simulink model "FMS"  (R2018b)
settings: configuration reference "fms_config" (kept outside this file)
values from neighbouring files (symbols this model uses):
  FMS_EXPORT = Simulink.Parameter(FMS_EXPORT_VALUE)    [fms_model_init.m]
  FMS_PARAM = Simulink.Parameter(FMS_PARAM_VALUE)    [fms_model_init.m]
undefined symbols (not defined in the file or in its folder): actuator_cmd, ax_cmd, ay_cmd, az_cmd, cmd_mask, ControlMode, ctrl_mode, DiscIntNeverNeededParam, ext_state, FMS_Cmd, FMS_CONST, home, mode, p_cmd, phi_cmd, PilotMode, psi_rate_cmd, q_cmd, r_cmd, reset, state, status, theta_cmd, throttle_cmd, timestamp, u_cmd, v_cmd, VehicleState, VehicleStatus, VTOLState, w_cmd, wp_consume, wp_current
libraries: simulink x141, FMT_Model_Lib x120, hdlsllib x13
(part 2 of 12)

== system FMS/FMS Commander/Commander/Arm/FW_Mode/SubMode ==
  In Bus Element{1..5} (5 alike) : Inport  PortName=FMS_In
  Action Port : ActionPort  InitializeStates=reset  ActionType=case
  Bus Selector : BusSelector  OutputSignals=vehicle_state
  Hold : Subsystem
      settings: UndoDeleteFcn=Stateflow.SLINSF.SimulinkMan.restorePreDeleteFcn  PreDeleteFcn=Stateflow.SLINSF.SimulinkMan.removePreDeleteFcn
  Land : Subsystem
      settings: UndoDeleteFcn=Stateflow.SLINSF.SimulinkMan.restorePreDeleteFcn  PreDeleteFcn=Stateflow.SLINSF.SimulinkMan.removePreDeleteFcn
  Merge : Merge  Inputs=5
  Return : Subsystem
      settings: UndoDeleteFcn=Stateflow.SLINSF.SimulinkMan.restorePreDeleteFcn  PreDeleteFcn=Stateflow.SLINSF.SimulinkMan.removePreDeleteFcn
  Switch Case : SwitchCase  CaseConditions={VehicleState.Takeoff, VehicleState.Land, VehicleState.Return,VehicleState.Hold}
  Takeoff : Subsystem
      settings: UndoDeleteFcn=Stateflow.SLINSF.SimulinkMan.restorePreDeleteFcn  PreDeleteFcn=Stateflow.SLINSF.SimulinkMan.removePreDeleteFcn
  Unknown : Subsystem  TreatAsAtomicUnit=on
  FMS_Out : Outport
  wires:
  Merge/1 -> FMS_Out/1
  In Bus Element1/1 -> Land/1(FMS_In)
  Land/1(FMS_Out) -> Merge/2
  Switch Case/2 -> Land/Action
  Switch Case/1 -> Takeoff/Action
  In Bus Element2/1 -> Takeoff/1(FMS_In)
  Takeoff/1(FMS_Out) -> Merge/1
  Switch Case/3 -> Return/Action
  In Bus Element3/1 -> Return/1(FMS_In)
  Return/1(FMS_Out) -> Merge/3
  Hold/1(FMS_Out) -> Merge/4
  In Bus Element4/1 -> Hold/1(FMS_In)
  Switch Case/4 -> Hold/Action
  Switch Case/5 -> Unknown/Action
  Unknown/1(FMS_Out) -> Merge/5
  In Bus Element5/1 -> Bus Selector/1
  Bus Selector/1 -> Switch Case/1  "<vehicle_state>"

== system FMS/FMS Commander/Commander/Arm/FW_Mode/Unknown ==
  Action Port : ActionPort  InitializeStates=reset  ActionType=default
  Bus Assignment : BusAssignment  AssignedSignals=reset,status,state,actuator_cmd
  Constant : Constant  Value=0  OutDataTypeStr=Bus: FMS_Out_Bus
  Constant1 : Constant  Value=VehicleStatus.Disarm
  Constant2 : Constant  OutDataTypeStr=Inherit: Inherit via back propagation
  Constant3 : Constant  Value=[1000;1000;1000;1000]  VectorParams1D=off  OutDataTypeStr=Inherit: Inherit via back propagation
  Constant4 : Constant  Value=zeros(12,1)  OutDataTypeStr=Inherit: Inherit via back propagation
  Constant5 : Constant  Value=VehicleState.Disarm
  Data Type Conversion : DataTypeConversion
  Data Type Conversion1 : DataTypeConversion
  Mux : Mux  Inputs=2
  FMS_Out : Outport
  wires:
  Mux/1 -> Bus Assignment/5
  Constant4/1 -> Mux/2
  Constant3/1 -> Mux/1
  Constant1/1 -> Data Type Conversion/1
  Constant2/1 -> Bus Assignment/2
  Bus Assignment/1 -> FMS_Out/1
  Constant/1 -> Bus Assignment/1
  Constant5/1 -> Data Type Conversion1/1
  Data Type Conversion/1 -> Bus Assignment/3
  Data Type Conversion1/1 -> Bus Assignment/4

== system FMS/FMS Commander/Commander/Arm/MC_Mode/Assist ==
  In Bus Element{1..5} (5 alike) : Inport  PortName=FMS_In
  Action Port : ActionPort  InitializeStates=reset  ActionType=case
  Acro : Subsystem
      settings: UndoDeleteFcn=Stateflow.SLINSF.SimulinkMan.restorePreDeleteFcn  PreDeleteFcn=Stateflow.SLINSF.SimulinkMan.removePreDeleteFcn
  Altitude : Subsystem
      settings: UndoDeleteFcn=Stateflow.SLINSF.SimulinkMan.restorePreDeleteFcn  PreDeleteFcn=Stateflow.SLINSF.SimulinkMan.removePreDeleteFcn
  Bus Selector : BusSelector  OutputSignals=vehicle_state
  Merge : Merge  Inputs=5
  Position : Subsystem
      settings: UndoDeleteFcn=Stateflow.SLINSF.SimulinkMan.restorePreDeleteFcn  PreDeleteFcn=Stateflow.SLINSF.SimulinkMan.removePreDeleteFcn
  Stabilize : Subsystem
      settings: UndoDeleteFcn=Stateflow.SLINSF.SimulinkMan.restorePreDeleteFcn  PreDeleteFcn=Stateflow.SLINSF.SimulinkMan.removePreDeleteFcn
  Switch Case : SwitchCase  CaseConditions={VehicleState.Acro,VehicleState.Stabilize,VehicleState.Altitude,VehicleState.Position}
  Unknown : Subsystem  TreatAsAtomicUnit=on
  FMS_Out : Outport
  wires:
  In Bus Element1/1 -> Position/1(FMS_In)
  Switch Case/4 -> Position/Action
  Switch Case/3 -> Altitude/Action
  In Bus Element2/1 -> Altitude/1(FMS_In)
  Switch Case/2 -> Stabilize/Action
  In Bus Element3/1 -> Stabilize/1(FMS_In)
  In Bus Element4/1 -> Acro/1(FMS_In)
  Switch Case/1 -> Acro/Action
  Acro/1(FMS_Out) -> Merge/1
  Stabilize/1(FMS_Out) -> Merge/2
  Altitude/1(FMS_Out) -> Merge/3
  Position/1(FMS_Out) -> Merge/4
  Merge/1 -> FMS_Out/1
  Unknown/1(FMS_Out) -> Merge/5
  Switch Case/5 -> Unknown/Action
  In Bus Element5/1 -> Bus Selector/1
  Bus Selector/1 -> Switch Case/1  "<vehicle_state>"

== system FMS/FMS Commander/Commander/Arm/MC_Mode/Auto ==
  In Bus Element6 : Inport  PortName=FMS_In
  In Bus Element1 : Inport  PortName=FMS_In
  In Bus Element2 : Inport  PortName=FMS_In
  Action Port : ActionPort  InitializeStates=reset  ActionType=case
  Bus Selector : BusSelector  OutputSignals=vehicle_state
  Merge : Merge  Inputs=3
  Mission : Subsystem
      settings: UndoDeleteFcn=Stateflow.SLINSF.SimulinkMan.restorePreDeleteFcn  PreDeleteFcn=Stateflow.SLINSF.SimulinkMan.removePreDeleteFcn
  Offboard : Subsystem
      settings: UndoDeleteFcn=Stateflow.SLINSF.SimulinkMan.restorePreDeleteFcn  PreDeleteFcn=Stateflow.SLINSF.SimulinkMan.removePreDeleteFcn
  Switch Case : SwitchCase  CaseConditions={VehicleState.Offboard,VehicleState.Mission}
  Unknown : Subsystem  TreatAsAtomicUnit=on
  FMS_Out : Outport
  wires:
  Merge/1 -> FMS_Out/1
  In Bus Element6/1 -> Offboard/1(FMS_In)
  Switch Case/1 -> Offboard/Action
  In Bus Element1/1 -> Mission/1(FMS_In)
  Switch Case/2 -> Mission/Action
  Offboard/1(FMS_Out) -> Merge/1
  Mission/1(FMS_Out) -> Merge/2
  Unknown/1(FMS_Out) -> Merge/3
  Switch Case/3 -> Unknown/Action
  In Bus Element2/1 -> Bus Selector/1
  Bus Selector/1 -> Switch Case/1  "<vehicle_state>"

== system FMS/FMS Commander/Commander/Arm/MC_Mode/Manual ==
  In Bus Element7 : Inport  PortName=FMS_In
  Action Port : ActionPort  InitializeStates=reset  ActionType=case
  Bus Assignment : BusAssignment  AssignedSignals=reset,status,state
  Constant : Constant  Value=0  OutDataTypeStr=Bus: FMS_Out_Bus
  Constant1 : Constant  Value=VehicleStatus.Disarm
  Constant2 : Constant  OutDataTypeStr=Inherit: Inherit via back propagation
  Constant5 : Constant  Value=VehicleState.Manual
  Data Type Conversion : DataTypeConversion
  Data Type Conversion1 : DataTypeConversion
  Terminator : Terminator
  FMS_Out : Outport
  wires:
  Data Type Conversion1/1 -> Bus Assignment/4
  Data Type Conversion/1 -> Bus Assignment/3
  Constant5/1 -> Data Type Conversion1/1
  Constant/1 -> Bus Assignment/1
  Bus Assignment/1 -> FMS_Out/1
  Constant2/1 -> Bus Assignment/2
  Constant1/1 -> Data Type Conversion/1
  In Bus Element7/1 -> Terminator/1

== system FMS/FMS Commander/Commander/Arm/MC_Mode/SubMode ==
  In Bus Element{1..5} (5 alike) : Inport  PortName=FMS_In
  Action Port : ActionPort  InitializeStates=reset  ActionType=case
  Bus Selector : BusSelector  OutputSignals=vehicle_state
  Hold : Subsystem
      settings: UndoDeleteFcn=Stateflow.SLINSF.SimulinkMan.restorePreDeleteFcn  PreDeleteFcn=Stateflow.SLINSF.SimulinkMan.removePreDeleteFcn
  Land : Subsystem
      settings: UndoDeleteFcn=Stateflow.SLINSF.SimulinkMan.restorePreDeleteFcn  PreDeleteFcn=Stateflow.SLINSF.SimulinkMan.removePreDeleteFcn
  Merge : Merge  Inputs=5
  Return : Subsystem
      settings: UndoDeleteFcn=Stateflow.SLINSF.SimulinkMan.restorePreDeleteFcn  PreDeleteFcn=Stateflow.SLINSF.SimulinkMan.removePreDeleteFcn
  Switch Case : SwitchCase  CaseConditions={VehicleState.Takeoff, VehicleState.Land, VehicleState.Return,VehicleState.Hold}
  Takeoff : Subsystem
      settings: UndoDeleteFcn=Stateflow.SLINSF.SimulinkMan.restorePreDeleteFcn  PreDeleteFcn=Stateflow.SLINSF.SimulinkMan.removePreDeleteFcn
  Unknown : Subsystem  TreatAsAtomicUnit=on
  FMS_Out : Outport
  wires:
  Merge/1 -> FMS_Out/1
  In Bus Element1/1 -> Land/1(FMS_In)
  Land/1(FMS_Out) -> Merge/2
  Switch Case/2 -> Land/Action
  Switch Case/1 -> Takeoff/Action
  In Bus Element2/1 -> Takeoff/1(FMS_In)
  Takeoff/1(FMS_Out) -> Merge/1
  Switch Case/3 -> Return/Action
  In Bus Element3/1 -> Return/1(FMS_In)
  Return/1(FMS_Out) -> Merge/3
  Hold/1(FMS_Out) -> Merge/4
  In Bus Element4/1 -> Hold/1(FMS_In)
  Switch Case/4 -> Hold/Action
  Switch Case/5 -> Unknown/Action
  Unknown/1(FMS_Out) -> Merge/5
  In Bus Element5/1 -> Bus Selector/1
  Bus Selector/1 -> Switch Case/1  "<vehicle_state>"

== system FMS/FMS Commander/Commander/Arm/MC_Mode/Unknown ==
  Action Port : ActionPort  InitializeStates=reset  ActionType=default
  Bus Assignment : BusAssignment  AssignedSignals=reset,status,state,actuator_cmd
  Constant : Constant  Value=0  OutDataTypeStr=Bus: FMS_Out_Bus
  Constant1 : Constant  Value=VehicleStatus.Disarm
  Constant2 : Constant  OutDataTypeStr=Inherit: Inherit via back propagation
  Constant3 : Constant  Value=[1000;1000;1000;1000]  VectorParams1D=off  OutDataTypeStr=Inherit: Inherit via back propagation
  Constant4 : Constant  Value=zeros(12,1)  OutDataTypeStr=Inherit: Inherit via back propagation
  Constant5 : Constant  Value=VehicleState.Disarm
  Data Type Conversion : DataTypeConversion
  Data Type Conversion1 : DataTypeConversion
  Mux : Mux  Inputs=2
  FMS_Out : Outport
  wires:
  Mux/1 -> Bus Assignment/5
  Constant4/1 -> Mux/2
  Constant3/1 -> Mux/1
  Constant1/1 -> Data Type Conversion/1
  Constant2/1 -> Bus Assignment/2
  Bus Assignment/1 -> FMS_Out/1
  Constant/1 -> Bus Assignment/1
  Constant5/1 -> Data Type Conversion1/1
  Data Type Conversion/1 -> Bus Assignment/3
  Data Type Conversion1/1 -> Bus Assignment/4

== system FMS/FMS Commander/Commander/Arm/BackwardTrans_Mode/Position Command/Controller ==
  motion_state : Inport
  In Bus Element : Inport  Port=2  PortName=FMS_In
  In Bus Element1 : Inport  Port=2  PortName=FMS_In
  Brake Control : Subsystem  TreatAsAtomicUnit=on
  Hold Control : Subsystem  TreatAsAtomicUnit=on
  Merge : Merge  Inputs=3
  Move Control : Subsystem  TreatAsAtomicUnit=on
  Saturation1 : Saturate  UpperLimit=FMS_PARAM.FW_ACC_Y_LIM  LowerLimit=-FMS_PARAM.FW_ACC_Y_LIM
  Switch Case : SwitchCase  CaseConditions={MotionState.Hold, MotionState.Brake, MotionState.Move}  ShowDefaultCase=off
  ay_cmd_mPs2 : Outport
  wires:
  Move Control/1(ay_cmd_mPs2) -> Merge/3
  Brake Control/1(ay_cmd_mPs2) -> Merge/2
  Hold Control/1(ay_cmd_mPs2) -> Merge/1
  In Bus Element/1 -> Hold Control/1(FMS_In)
  Switch Case/3 -> Move Control/Action
  Switch Case/2 -> Brake Control/Action
  Switch Case/1 -> Hold Control/Action
  motion_state/1 -> Switch Case/1
  Saturation1/1 -> ay_cmd_mPs2/1
  Merge/1 -> Saturation1/1
  In Bus Element1/1 -> Move Control/1(FMS_In)

== system FMS/FMS Commander/Commander/Arm/BackwardTrans_Mode/Position Command/Detect Movement ==
  FMS_In : Inport
  Abs : Abs
  Abs1 : Abs
  Abs2 : Abs
  Bus Selector1 : BusSelector  OutputSignals=Pilot_Cmd.stick_roll,Pilot_Cmd.stick_yaw
  Bus Selector2 : BusSelector  OutputSignals=INS_Out.psi,INS_Out.vn,INS_Out.ve,INS_Out.vd
  Compare To Constant : simulink/Logic and Bit Operations/Compare To Constant  relop=>  const=FMS_PARAM.ROLL_DZ  OutDataTypeStr=boolean
  Compare To Constant1 : simulink/Logic and Bit Operations/Compare To Constant  relop=>  const=FMS_PARAM.YAW_DZ  OutDataTypeStr=boolean
  Logical Operator : Logic  Operator=OR  AllPortsSameDT=off  OutDataTypeStr=boolean
  Motion State : Stateflow chart  TreatAsAtomicUnit=on
  Multiply : Product  Multiplication=Matrix(*)
  Mux : Mux  Inputs=3
  Psi To DCM : FMT_Model_Lib/Transformation/Psi To DCM
      settings: SourceProductName=FMT Toolbox
  Selector : Selector  InputPortWidth=3  IndexOptions=Index vector (dialog)  Indices=1  OutputSizes=1
  motion_state : Outport
  wires:
  FMS_In/1 -> Bus Selector2/1, Bus Selector1/1
  Abs1/1 -> Compare To Constant/1
  Motion State/1(state) -> motion_state/1
  Abs/1 -> Motion State/2(speed)
  Bus Selector1/1 -> Abs1/1  "<stick_roll>"
  Bus Selector2/1 -> Psi To DCM/1  "<psi>"
  Bus Selector2/2 -> Mux/1  "<vn>"
  Bus Selector2/3 -> Mux/2  "<ve>"
  Bus Selector2/4 -> Mux/3  "<vd>"
  Psi To DCM/1 -> Multiply/1
  Multiply/1 -> Selector/1
  Selector/1 -> Abs/1
  Mux/1 -> Multiply/2
  Bus Selector1/2 -> Abs2/1  "<stick_yaw>"
  Abs2/1 -> Compare To Constant1/1
  Compare To Constant/1 -> Logical Operator/1
  Compare To Constant1/1 -> Logical Operator/2
  Logical Operator/1 -> Motion State/1(motion_req)

== system FMS/FMS Commander/Commander/Arm/BackwardTrans_Mode/mapping/DeadZone ==
  u : Inport
  Dead Zone : DeadZone  LowerValue=-th  UpperValue=th  SaturateOnIntegerOverflow=on
  Gain : Gain  Gain=1/(1-th)
  y : Outport
  wires:
  Gain/1 -> y/1
  Dead Zone/1 -> Gain/1
  u/1 -> Dead Zone/1

== system FMS/FMS Commander/Commander/Arm/BackwardTrans_Mode/mapping/DeadZone1 ==
  u : Inport
  Dead Zone : DeadZone  LowerValue=-th  UpperValue=th  SaturateOnIntegerOverflow=on
  Gain : Gain  Gain=1/(1-th)
  y : Outport
  wires:
  u/1 -> Dead Zone/1
  Dead Zone/1 -> Gain/1
  Gain/1 -> y/1

== system FMS/FMS Commander/Commander/Arm/BackwardTrans_Mode/mapping/DeadZone2 ==
  u : Inport
  Dead Zone : DeadZone  LowerValue=-th  UpperValue=th  SaturateOnIntegerOverflow=on
  Gain : Gain  Gain=1/(1-th)
  y : Outport
  wires:
  Gain/1 -> y/1
  Dead Zone/1 -> Gain/1
  u/1 -> Dead Zone/1

== system FMS/FMS Commander/Commander/Arm/BackwardTrans_Mode/mapping/TD ==
  v : Inport
  Integrator : DiscreteIntegrator  SampleTime=-1  ICPrevOutput=DiscIntNeverNeededParam  ICPrevScaledInput=DiscIntNeverNeededParam
  Integrator1 : DiscreteIntegrator  SampleTime=-1  ICPrevOutput=DiscIntNeverNeededParam  ICPrevScaledInput=DiscIntNeverNeededParam
  Signal Copy : SignalConversion  OverrideOpt=off
  Subtract : Sum  Inputs=+-
  "fhan " : Subsystem  mask{r0=4*9.806, h0=0.1}
      mask DialogControl ParameterGroupVar Prompt: fhan(v1,v2,r0,h0)
  v1 : Outport
  wires:
  "fhan "/1(fhan) -> Integrator/1
  Subtract/1 -> "fhan "/1(v1)
  Integrator/1 -> Integrator1/1, "fhan "/2(v2)  "v2"
  v/1 -> Subtract/2
  Integrator1/1 -> Subtract/1, Signal Copy/1
  Signal Copy/1 -> v1/1

== system FMS/FMS Commander/Commander/Arm/BackwardTrans_Mode/mapping/TD1 ==
  v : Inport
  Integrator : DiscreteIntegrator  SampleTime=-1  ICPrevOutput=DiscIntNeverNeededParam  ICPrevScaledInput=DiscIntNeverNeededParam
  Integrator1 : DiscreteIntegrator  SampleTime=-1  ICPrevOutput=DiscIntNeverNeededParam  ICPrevScaledInput=DiscIntNeverNeededParam
  Signal Copy : SignalConversion  OverrideOpt=off
  Subtract : Sum  Inputs=+-
  "fhan " : Subsystem  mask{r0=5*pi, h0=0.02}
      mask DialogControl ParameterGroupVar Prompt: fhan(v1,v2,r0,h0)
  v1 : Outport
  wires:
  "fhan "/1(fhan) -> Integrator/1
  Subtract/1 -> "fhan "/1(v1)
  Integrator/1 -> Integrator1/1, "fhan "/2(v2)  "v2"
  v/1 -> Subtract/2
  Integrator1/1 -> Subtract/1, Signal Copy/1
  Signal Copy/1 -> v1/1

== system FMS/FMS Commander/Commander/Arm/BackwardTrans_Mode/mapping/TD2 ==
  v : Inport
  Integrator : DiscreteIntegrator  SampleTime=-1  ICPrevOutput=DiscIntNeverNeededParam  ICPrevScaledInput=DiscIntNeverNeededParam
  Integrator1 : DiscreteIntegrator  SampleTime=-1  ICPrevOutput=DiscIntNeverNeededParam  ICPrevScaledInput=DiscIntNeverNeededParam
  Signal Copy : SignalConversion  OverrideOpt=off
  Subtract : Sum  Inputs=+-
  "fhan " : Subsystem  mask{r0=4*9.806, h0=0.1}
      mask DialogControl ParameterGroupVar Prompt: fhan(v1,v2,r0,h0)
  v1 : Outport
  wires:
  Signal Copy/1 -> v1/1
  Integrator1/1 -> Signal Copy/1, Subtract/1
  v/1 -> Subtract/2
  Integrator/1 -> "fhan "/2(v2), Integrator1/1  "v2"
  Subtract/1 -> "fhan "/1(v1)
  "fhan "/1(fhan) -> Integrator/1

== system FMS/FMS Commander/Commander/Arm/FW_Mode/Assist/Altitude ==
  In Bus Element1 : Inport  PortName=FMS_In
  Action Port : ActionPort  InitializeStates=reset  ActionType=case
      settings: CopyFcn=Stateflow.SLINSF.SimulinkMan.removeBlockPreDeleteFcn
  Altitude Command : Subsystem
  Attitude Command : Subsystem
  Bus Assignment : BusAssignment  AssignedSignals=status,state,ctrl_mode,phi_cmd,psi_rate_cmd,u_cmd,w_cmd
  Constant : Constant  Value=0  OutDataTypeStr=Bus: FMS_Out_Bus
  Constant1 : Constant  Value=VehicleState.Altitude
  Constant2 : Constant  Value=ControlMode.ALTCTL
  Constant5 : Constant  Value=VehicleStatus.Arm
  Data Type Conversion1 : DataTypeConversion
  Data Type Conversion2 : DataTypeConversion
  Data Type Conversion3 : DataTypeConversion
  Heading Command : Subsystem
  Speed Command : Subsystem
  FMS_Out : Outport
  wires:
  Constant5/1 -> Data Type Conversion1/1
  Constant/1 -> Bus Assignment/1
  Altitude Command/1(w_cmd_mPs) -> Bus Assignment/8
  Attitude Command/1(phi_cmd_radPs) -> Bus Assignment/5
  Bus Assignment/1 -> FMS_Out/1
  Data Type Conversion1/1 -> Bus Assignment/2
  Constant1/1 -> Data Type Conversion2/1
  Data Type Conversion2/1 -> Bus Assignment/3
  Data Type Conversion3/1 -> Bus Assignment/4
  Constant2/1 -> Data Type Conversion3/1
  In Bus Element1/1 -> Heading Command/1(FMS_In), Attitude Command/1(FMS_In), Speed Command/1(FMS_In), Altitude Command/1(FMS_In)
  Speed Command/1(u_cmd_mPs) -> Bus Assignment/7
  Heading Command/1(psi_rate_cmd_radPs) -> Bus Assignment/6

== system FMS/FMS Commander/Commander/Arm/FW_Mode/Assist/Position ==
  FMS_In : Inport
  Action Port : ActionPort  InitializeStates=reset  ActionType=case
      settings: CopyFcn=Stateflow.SLINSF.SimulinkMan.removeBlockPreDeleteFcn
  Altitude Command : Subsystem
  Bus Assignment : BusAssignment  AssignedSignals=status,state,ctrl_mode,psi_rate_cmd,u_cmd,ay_cmd,w_cmd
  Constant : Constant  Value=0  OutDataTypeStr=Bus: FMS_Out_Bus
  Constant1 : Constant  Value=VehicleState.Position
  Constant2 : Constant  Value=ControlMode.POSCTL
  Constant5 : Constant  Value=VehicleStatus.Arm
  Data Type Conversion : DataTypeConversion
  Data Type Conversion1 : DataTypeConversion
  Data Type Conversion2 : DataTypeConversion
  Heading Command : Subsystem
  Position Command : Subsystem
  Speed Command : Subsystem
  FMS_Out : Outport
  wires:
  Bus Assignment/1 -> FMS_Out/1
  Altitude Command/1(w_cmd_mPs) -> Bus Assignment/8
  Constant/1 -> Bus Assignment/1
  Constant5/1 -> Data Type Conversion/1
  Position Command/1(ay_cmd_mPs2) -> Bus Assignment/7
  Data Type Conversion/1 -> Bus Assignment/2
  Constant1/1 -> Data Type Conversion1/1
  Data Type Conversion1/1 -> Bus Assignment/3
  Constant2/1 -> Data Type Conversion2/1
  Data Type Conversion2/1 -> Bus Assignment/4
  FMS_In/1 -> Altitude Command/1(FMS_In), Position Command/1(FMS_In), Heading Command/1(FMS_In), Speed Command/1(FMS_In)
  Speed Command/1(u_cmd_mPs) -> Bus Assignment/6
  Heading Command/1(psi_rate_cmd_radPs) -> Bus Assignment/5

== system FMS/FMS Commander/Commander/Arm/FW_Mode/Assist/Stabilize ==
  FMS_In : Inport
  Action Port : ActionPort  InitializeStates=reset  ActionType=case
      settings: CopyFcn=Stateflow.SLINSF.SimulinkMan.removeBlockPreDeleteFcn
  Attitude Command : Subsystem
  Bus Assignment : BusAssignment  AssignedSignals=status,state,ctrl_mode,phi_cmd,theta_cmd,psi_rate_cmd,throttle_cmd
  Constant : Constant  Value=0  OutDataTypeStr=Bus: FMS_Out_Bus
  Constant1 : Constant  Value=VehicleState.Stabilize
  Constant2 : Constant  Value=ControlMode.Stabilize
  Constant5 : Constant  Value=VehicleStatus.Arm
  Data Type Conversion : DataTypeConversion
  Data Type Conversion1 : DataTypeConversion
  Data Type Conversion2 : DataTypeConversion
  Heading Command : Subsystem
  Throttle Command : Subsystem
  FMS_Out : Outport
  wires:
  Constant5/1 -> Data Type Conversion/1
  Constant/1 -> Bus Assignment/1
  Attitude Command/1(phi_cmd_radPs) -> Bus Assignment/5
  Throttle Command/1(throttle_cmd) -> Bus Assignment/8
  Attitude Command/2(theta_cmd_radPs) -> Bus Assignment/6
  FMS_In/1 -> Heading Command/1(FMS_In), Throttle Command/1(FMS_In), Attitude Command/1(FMS_In)
  Bus Assignment/1 -> FMS_Out/1
  Data Type Conversion/1 -> Bus Assignment/2
  Constant1/1 -> Data Type Conversion1/1
  Data Type Conversion1/1 -> Bus Assignment/3
  Constant2/1 -> Data Type Conversion2/1
  Data Type Conversion2/1 -> Bus Assignment/4
  Heading Command/1(psi_rate_cmd_radPs) -> Bus Assignment/7

== system FMS/FMS Commander/Commander/Arm/FW_Mode/Assist/Unknown ==
  Action Port : ActionPort  InitializeStates=reset  ActionType=default
  Bus Assignment : BusAssignment  AssignedSignals=reset,status,state,actuator_cmd
  Constant : Constant  Value=0  OutDataTypeStr=Bus: FMS_Out_Bus
  Constant1 : Constant  Value=VehicleStatus.Disarm
  Constant2 : Constant  OutDataTypeStr=Inherit: Inherit via back propagation
  Constant3 : Constant  Value=[1000;1000;1000;1000]  VectorParams1D=off  OutDataTypeStr=Inherit: Inherit via back propagation
  Constant4 : Constant  Value=zeros(12,1)  OutDataTypeStr=Inherit: Inherit via back propagation
  Constant5 : Constant  Value=VehicleState.Disarm
  Data Type Conversion : DataTypeConversion
  Data Type Conversion1 : DataTypeConversion
  Mux : Mux  Inputs=2
  FMS_Out : Outport
  wires:
  Mux/1 -> Bus Assignment/5
  Constant4/1 -> Mux/2
  Constant3/1 -> Mux/1
  Constant1/1 -> Data Type Conversion/1
  Constant2/1 -> Bus Assignment/2
  Bus Assignment/1 -> FMS_Out/1
  Constant/1 -> Bus Assignment/1
  Constant5/1 -> Data Type Conversion1/1
  Data Type Conversion/1 -> Bus Assignment/3
  Data Type Conversion1/1 -> Bus Assignment/4

== system FMS/FMS Commander/Commander/Arm/FW_Mode/Auto/Mission ==
  FMS_In : Inport
  Action Port : ActionPort  InitializeStates=reset  ActionType=case
      settings: CopyFcn=Stateflow.SLINSF.SimulinkMan.removeBlockPreDeleteFcn
  Bus Selector : BusSelector  OutputSignals=wp_index
  Detect Change : simulink/Logic and Bit Operations/Detect Change  vinit=0  OutDataTypeStr=boolean
  Mission_SubSystem : Subsystem  TreatAsAtomicUnit=on
  FMS_Out : Outport
  wires:
  Mission_SubSystem/1(FMS_Out) -> FMS_Out/1
  FMS_In/1 -> Bus Selector/1, Mission_SubSystem/1(FMS_In)
  Bus Selector/1 -> Detect Change/1  "<wp_index>"
  Detect Change/1 -> Mission_SubSystem/Reset

== system FMS/FMS Commander/Commander/Arm/FW_Mode/Auto/Offboard ==
  FMS_In : Inport
  Action Port : ActionPort  InitializeStates=reset  ActionType=case
      settings: CopyFcn=Stateflow.SLINSF.SimulinkMan.removeBlockPreDeleteFcn
  Bus Assignment : BusAssignment  AssignedSignals=status,state
  Constant : Constant  Value=0  OutDataTypeStr=Bus: FMS_Out_Bus
  Constant1 : Constant  Value=VehicleStatus.Disarm
  Constant2 : Constant  Value=VehicleState.Offboard
  Data Type Conversion : DataTypeConversion
  Data Type Conversion1 : DataTypeConversion
  Terminator : Terminator
  FMS_Out : Outport
  wires:
  Bus Assignment/1 -> FMS_Out/1
  Constant/1 -> Bus Assignment/1
  FMS_In/1 -> Terminator/1
  Constant1/1 -> Data Type Conversion/1
  Data Type Conversion/1 -> Bus Assignment/2
  Constant2/1 -> Data Type Conversion1/1
  Data Type Conversion1/1 -> Bus Assignment/3

== system FMS/FMS Commander/Commander/Arm/FW_Mode/Auto/Unknown ==
  Action Port : ActionPort  InitializeStates=reset  ActionType=default
  Bus Assignment : BusAssignment  AssignedSignals=reset,status,state,actuator_cmd
  Constant : Constant  Value=0  OutDataTypeStr=Bus: FMS_Out_Bus
  Constant1 : Constant  Value=VehicleStatus.Disarm
  Constant2 : Constant  OutDataTypeStr=Inherit: Inherit via back propagation
  Constant3 : Constant  Value=[1000;1000;1000;1000]  VectorParams1D=off  OutDataTypeStr=Inherit: Inherit via back propagation
  Constant4 : Constant  Value=zeros(12,1)  OutDataTypeStr=Inherit: Inherit via back propagation
  Constant5 : Constant  Value=VehicleState.Disarm
  Data Type Conversion : DataTypeConversion
  Data Type Conversion1 : DataTypeConversion
  Mux : Mux  Inputs=2
  FMS_Out : Outport
  wires:
  Mux/1 -> Bus Assignment/5
  Constant4/1 -> Mux/2
  Constant3/1 -> Mux/1
  Constant1/1 -> Data Type Conversion/1
  Constant2/1 -> Bus Assignment/2
  Bus Assignment/1 -> FMS_Out/1
  Constant/1 -> Bus Assignment/1
  Constant5/1 -> Data Type Conversion1/1
  Data Type Conversion/1 -> Bus Assignment/3
  Data Type Conversion1/1 -> Bus Assignment/4

== system FMS/FMS Commander/Commander/Arm/FW_Mode/Manual/DeadZone ==
  u : Inport
  Dead Zone : DeadZone  LowerValue=-th  UpperValue=th  SaturateOnIntegerOverflow=on
  Gain : Gain  Gain=1/(1-th)
  y : Outport
  wires:
  Gain/1 -> y/1
  Dead Zone/1 -> Gain/1
  u/1 -> Dead Zone/1

== system FMS/FMS Commander/Commander/Arm/FW_Mode/Manual/DeadZone1 ==
  u : Inport
  Dead Zone : DeadZone  LowerValue=-th  UpperValue=th  SaturateOnIntegerOverflow=on
  Gain : Gain  Gain=1/(1-th)
  y : Outport
  wires:
  u/1 -> Dead Zone/1
  Dead Zone/1 -> Gain/1
  Gain/1 -> y/1

== system FMS/FMS Commander/Commander/Arm/FW_Mode/Manual/DeadZone2 ==
  u : Inport
  Dead Zone : DeadZone  LowerValue=-th  UpperValue=th  SaturateOnIntegerOverflow=on
  Gain : Gain  Gain=1/(1-th)
  y : Outport
  wires:
  Gain/1 -> y/1
  Dead Zone/1 -> Gain/1
  u/1 -> Dead Zone/1

== system FMS/FMS Commander/Commander/Arm/FW_Mode/Manual/DeadZone3 ==
  u : Inport
  Dead Zone : DeadZone  LowerValue=-th  UpperValue=th  SaturateOnIntegerOverflow=on
  Gain : Gain  Gain=1/(1-th)
  y : Outport
  wires:
  u/1 -> Dead Zone/1
  Dead Zone/1 -> Gain/1
  Gain/1 -> y/1

== system FMS/FMS Commander/Commander/Arm/FW_Mode/SubMode/Hold ==
  FMS_In : Inport
  Action Port : ActionPort  InitializeStates=reset  ActionType=case
      settings: CopyFcn=Stateflow.SLINSF.SimulinkMan.removeBlockPreDeleteFcn
  Altitude_Hold : Subsystem
  Bus Assignment : BusAssignment  AssignedSignals=status,state,ctrl_mode,u_cmd,ay_cmd,w_cmd
  Constant : Constant  Value=0  OutDataTypeStr=Bus: FMS_Out_Bus
  Constant1 : Constant  Value=VehicleState.Hold
  Constant2 : Constant  Value=ControlMode.POSCTL
  Constant3 : Constant  Value=15  OutDataTypeStr=single
  Constant5 : Constant  Value=VehicleStatus.Arm
  Data Type Conversion : DataTypeConversion
  Data Type Conversion1 : DataTypeConversion
  Data Type Conversion2 : DataTypeConversion
  Loiter_Control : Subsystem
  FMS_Out : Outport
  wires:
  Bus Assignment/1 -> FMS_Out/1
  Altitude_Hold/1(w_cmd_mPs) -> Bus Assignment/7
  Constant/1 -> Bus Assignment/1
  Constant5/1 -> Data Type Conversion/1
  Data Type Conversion/1 -> Bus Assignment/2
  Constant1/1 -> Data Type Conversion1/1
  Data Type Conversion1/1 -> Bus Assignment/3
  Constant2/1 -> Data Type Conversion2/1
  Data Type Conversion2/1 -> Bus Assignment/4
  FMS_In/1 -> Altitude_Hold/1(FMS_In), Loiter_Control/1(FMS_In)
  Loiter_Control/1(ay_cmd_mPs2) -> Bus Assignment/6
  Constant3/1 -> Bus Assignment/5

== system FMS/FMS Commander/Commander/Arm/FW_Mode/SubMode/Land ==
  FMS_In : Inport
  Action Port : ActionPort  InitializeStates=reset  ActionType=case
      settings: CopyFcn=Stateflow.SLINSF.SimulinkMan.removeBlockPreDeleteFcn
  Bus Assignment1 : BusAssignment  AssignedSignals=status,state,ctrl_mode,psi_rate_cmd,u_cmd,v_cmd,w_cmd
  Constant : Constant  Value=0  OutDataTypeStr=Inherit: Inherit via back propagation
  Constant1 : Constant  Value=0  OutDataTypeStr=Bus: FMS_Out_Bus
  Constant2 : Constant  Value=ControlMode.POSCTL
  Constant3 : Constant  Value=VehicleState.Land
  Constant4 : Constant  Value=0.5  OutDataTypeStr=Inherit: Inherit via back propagation
  Constant5 : Constant  Value=0  OutDataTypeStr=Inherit: Inherit via back propagation
  Constant6 : Constant  Value=VehicleStatus.Arm
  Constant7 : Constant  Value=0  OutDataTypeStr=Inherit: Inherit via back propagation
  Data Type Conversion : DataTypeConversion
  Data Type Conversion1 : DataTypeConversion
  Data Type Conversion2 : DataTypeConversion
  Terminator : Terminator
  FMS_Out : Outport
  wires:
  Bus Assignment1/1 -> FMS_Out/1
  Constant1/1 -> Bus Assignment1/1
  FMS_In/1 -> Terminator/1
  Constant4/1 -> Bus Assignment1/8
  Constant/1 -> Bus Assignment1/5
  Constant2/1 -> Data Type Conversion2/1
  Constant6/1 -> Data Type Conversion/1
  Data Type Conversion/1 -> Bus Assignment1/2
  Constant3/1 -> Data Type Conversion1/1
  Data Type Conversion1/1 -> Bus Assignment1/3
  Data Type Conversion2/1 -> Bus Assignment1/4
  Constant5/1 -> Bus Assignment1/6
  Constant7/1 -> Bus Assignment1/7

== system FMS/FMS Commander/Commander/Arm/FW_Mode/SubMode/Return ==
  FMS_In : Inport
  Action Port : ActionPort  InitializeStates=reset  ActionType=case
      settings: CopyFcn=Stateflow.SLINSF.SimulinkMan.removeBlockPreDeleteFcn
  Altitude Control : Subsystem
  Bus Assignment1 : BusAssignment  AssignedSignals=status,state,ctrl_mode,u_cmd,ay_cmd,w_cmd
  Constant1 : Constant  Value=VehicleState.Return
  Constant2 : Constant  Value=0  OutDataTypeStr=Bus: FMS_Out_Bus
  Constant3 : Constant  Value=ControlMode.POSCTL
  Constant4 : Constant  Value=FMS_PARAM.FW_CRUISE_SPEED
  Constant6 : Constant  Value=VehicleStatus.Arm
  Data Type Conversion : DataTypeConversion
  Data Type Conversion1 : DataTypeConversion
  Data Type Conversion2 : DataTypeConversion
  Position Command : Subsystem
  FMS_Out : Outport
  wires:
  Constant3/1 -> Data Type Conversion2/1
  Constant2/1 -> Bus Assignment1/1
  Bus Assignment1/1 -> FMS_Out/1
  Data Type Conversion/1 -> Bus Assignment1/2
  Constant6/1 -> Data Type Conversion/1
  Data Type Conversion1/1 -> Bus Assignment1/3
  Data Type Conversion2/1 -> Bus Assignment1/4
  Constant1/1 -> Data Type Conversion1/1
  FMS_In/1 -> Altitude Control/1(FMS_In), Position Command/1(FMS_In)
  Position Command/1(ay_cmd_mPs2) -> Bus Assignment1/6
  Constant4/1 -> Bus Assignment1/5
  Altitude Control/1(w_cmd_mPs) -> Bus Assignment1/7

== system FMS/FMS Commander/Commander/Arm/FW_Mode/SubMode/Takeoff ==
  FMS_In : Inport
  Action Port : ActionPort  InitializeStates=reset  ActionType=case
      settings: CopyFcn=Stateflow.SLINSF.SimulinkMan.removeBlockPreDeleteFcn
  Altitude Control : Subsystem
  Bus Assignment : BusAssignment  AssignedSignals=status,state,ctrl_mode,u_cmd,ay_cmd,w_cmd
  Constant : Constant  Value=0  OutDataTypeStr=Bus: FMS_Out_Bus
  Constant1 : Constant  Value=VehicleStatus.Arm
  Constant2 : Constant  Value=VehicleState.Takeoff
  Constant3 : Constant  Value=ControlMode.POSCTL
  Constant4 : Constant  Value=FMS_PARAM.FW_CRUISE_SPEED
  Data Type Conversion : DataTypeConversion
  Data Type Conversion1 : DataTypeConversion
  Data Type Conversion2 : DataTypeConversion
  Position Command : Subsystem
  FMS_Out : Outport
  wires:
  Data Type Conversion1/1 -> Bus Assignment/3
  Bus Assignment/1 -> FMS_Out/1
  Constant1/1 -> Data Type Conversion/1
  Constant/1 -> Bus Assignment/1
  Data Type Conversion2/1 -> Bus Assignment/4
  FMS_In/1 -> Altitude Control/1(FMS_In), Position Command/1(FMS_In)
  Data Type Conversion/1 -> Bus Assignment/2
  Constant3/1 -> Data Type Conversion2/1
  Position Command/1(ay_cmd_mPs2) -> Bus Assignment/6
  Constant2/1 -> Data Type Conversion1/1
  Altitude Control/1(w_cmd_mPs) -> Bus Assignment/7
  Constant4/1 -> Bus Assignment/5

== system FMS/FMS Commander/Commander/Arm/FW_Mode/SubMode/Unknown ==
  Action Port : ActionPort  InitializeStates=reset  ActionType=default
  Bus Assignment : BusAssignment  AssignedSignals=reset,status,state,actuator_cmd
  Constant : Constant  Value=0  OutDataTypeStr=Bus: FMS_Out_Bus
  Constant1 : Constant  Value=VehicleStatus.Disarm
  Constant2 : Constant  OutDataTypeStr=Inherit: Inherit via back propagation
  Constant3 : Constant  Value=[1000;1000;1000;1000]  VectorParams1D=off  OutDataTypeStr=Inherit: Inherit via back propagation
  Constant4 : Constant  Value=zeros(12,1)  OutDataTypeStr=Inherit: Inherit via back propagation
  Constant5 : Constant  Value=VehicleState.Disarm
  Data Type Conversion : DataTypeConversion
  Data Type Conversion1 : DataTypeConversion
  Mux : Mux  Inputs=2
  FMS_Out : Outport
  wires:
  Mux/1 -> Bus Assignment/5
  Constant4/1 -> Mux/2
  Constant3/1 -> Mux/1
  Constant1/1 -> Data Type Conversion/1
  Constant2/1 -> Bus Assignment/2
  Bus Assignment/1 -> FMS_Out/1
  Constant/1 -> Bus Assignment/1
  Constant5/1 -> Data Type Conversion1/1
  Data Type Conversion/1 -> Bus Assignment/3
  Data Type Conversion1/1 -> Bus Assignment/4

== system FMS/FMS Commander/Commander/Arm/MC_Mode/Assist/Acro ==
  FMS_In : Inport
  Action Port : ActionPort  InitializeStates=reset  ActionType=case
      settings: CopyFcn=Stateflow.SLINSF.SimulinkMan.removeBlockPreDeleteFcn
  Angular Rate Command : Subsystem
  Bus Assignment : BusAssignment  AssignedSignals=status,state,ctrl_mode,p_cmd,q_cmd,r_cmd,throttle_cmd
  Constant : Constant  Value=0  OutDataTypeStr=Bus: FMS_Out_Bus
  Constant1 : Constant  Value=VehicleState.Acro
  Constant2 : Constant  Value=ControlMode.Acro
  Constant5 : Constant  Value=VehicleStatus.Arm
  Data Type Conversion : DataTypeConversion
  Data Type Conversion1 : DataTypeConversion
  Data Type Conversion2 : DataTypeConversion
  Throttle Command : Subsystem
  FMS_Out : Outport
  wires:
  Data Type Conversion2/1 -> Bus Assignment/4
  Constant2/1 -> Data Type Conversion2/1
  Data Type Conversion1/1 -> Bus Assignment/3
  Constant1/1 -> Data Type Conversion1/1
  Data Type Conversion/1 -> Bus Assignment/2
  Bus Assignment/1 -> FMS_Out/1
  Throttle Command/1(throttle_cmd) -> Bus Assignment/8
  Constant/1 -> Bus Assignment/1
  Constant5/1 -> Data Type Conversion/1
  Angular Rate Command/1(p_cmd_radPs) -> Bus Assignment/5
  Angular Rate Command/2(q_cmd_radPs) -> Bus Assignment/6
  Angular Rate Command/3(r_cmd_radPs) -> Bus Assignment/7
  FMS_In/1 -> Throttle Command/1(FMS_In), Angular Rate Command/1(FMS_In)

== system FMS/FMS Commander/Commander/Arm/MC_Mode/Assist/Altitude ==
  In Bus Element1 : Inport  PortName=FMS_In
  Action Port : ActionPort  InitializeStates=reset  ActionType=case
      settings: CopyFcn=Stateflow.SLINSF.SimulinkMan.removeBlockPreDeleteFcn
  Altitude Command : Subsystem
  Attitude Command : Subsystem
  Bus Assignment : BusAssignment  AssignedSignals=status,state,ctrl_mode,phi_cmd,theta_cmd,psi_rate_cmd,w_cmd
  Constant : Constant  Value=0  OutDataTypeStr=Bus: FMS_Out_Bus
  Constant1 : Constant  Value=VehicleState.Altitude
  Constant2 : Constant  Value=ControlMode.ALTCTL
  Constant5 : Constant  Value=VehicleStatus.Arm
  Data Type Conversion1 : DataTypeConversion
  Data Type Conversion2 : DataTypeConversion
  Data Type Conversion3 : DataTypeConversion
  Heading Command : Subsystem
  FMS_Out : Outport
  wires:
  Constant5/1 -> Data Type Conversion1/1
  Constant/1 -> Bus Assignment/1
  Heading Command/1(psi_rate_cmd_radPs) -> Bus Assignment/7
  Altitude Command/1(w_cmd_mPs) -> Bus Assignment/8
  Attitude Command/1(phi_cmd_radPs) -> Bus Assignment/5
  Attitude Command/2(theta_cmd_radPs) -> Bus Assignment/6
  Bus Assignment/1 -> FMS_Out/1
  Data Type Conversion1/1 -> Bus Assignment/2
  Constant1/1 -> Data Type Conversion2/1
  Data Type Conversion2/1 -> Bus Assignment/3
  Data Type Conversion3/1 -> Bus Assignment/4
  Constant2/1 -> Data Type Conversion3/1
  In Bus Element1/1 -> Heading Command/1(FMS_In), Altitude Command/1(FMS_In), Attitude Command/1(FMS_In)

== system FMS/FMS Commander/Commander/Arm/MC_Mode/Assist/Position ==
  FMS_In : Inport
  Action Port : ActionPort  InitializeStates=reset  ActionType=case
      settings: CopyFcn=Stateflow.SLINSF.SimulinkMan.removeBlockPreDeleteFcn
  Altitude Command : Subsystem
  Bus Assignment : BusAssignment  AssignedSignals=status,state,ctrl_mode,psi_rate_cmd,u_cmd,v_cmd,w_cmd
  Constant : Constant  Value=0  OutDataTypeStr=Bus: FMS_Out_Bus
  Constant1 : Constant  Value=VehicleState.Position
  Constant2 : Constant  Value=ControlMode.POSCTL
  Constant5 : Constant  Value=VehicleStatus.Arm
  Data Type Conversion : DataTypeConversion
  Data Type Conversion1 : DataTypeConversion
  Data Type Conversion2 : DataTypeConversion
  Heading Command : Subsystem
  Position Command : Subsystem
  FMS_Out : Outport
  wires:
  Bus Assignment/1 -> FMS_Out/1
  Altitude Command/1(w_cmd_mPs) -> Bus Assignment/8
  Constant/1 -> Bus Assignment/1
  Position Command/1(u_cmd_mPs) -> Bus Assignment/6
  Constant5/1 -> Data Type Conversion/1
  Position Command/2(v_cmd_mPs) -> Bus Assignment/7
  Heading Command/1(psi_rate_cmd_radPs) -> Bus Assignment/5
  Data Type Conversion/1 -> Bus Assignment/2
  Constant1/1 -> Data Type Conversion1/1
  Data Type Conversion1/1 -> Bus Assignment/3
  Constant2/1 -> Data Type Conversion2/1
  Data Type Conversion2/1 -> Bus Assignment/4
  FMS_In/1 -> Heading Command/1(FMS_In), Altitude Command/1(FMS_In), Position Command/1(FMS_In)

== system FMS/FMS Commander/Commander/Arm/MC_Mode/Assist/Stabilize ==
  FMS_In : Inport
  Action Port : ActionPort  InitializeStates=reset  ActionType=case
      settings: CopyFcn=Stateflow.SLINSF.SimulinkMan.removeBlockPreDeleteFcn
  Attitude Command : Subsystem
  Bus Assignment : BusAssignment  AssignedSignals=status,state,ctrl_mode,phi_cmd,theta_cmd,psi_rate_cmd,throttle_cmd
  Constant : Constant  Value=0  OutDataTypeStr=Bus: FMS_Out_Bus
  Constant1 : Constant  Value=VehicleState.Stabilize
  Constant2 : Constant  Value=ControlMode.Stabilize
  Constant5 : Constant  Value=VehicleStatus.Arm
  Data Type Conversion : DataTypeConversion
  Data Type Conversion1 : DataTypeConversion
  Data Type Conversion2 : DataTypeConversion
  Heading Command : Subsystem
  Throttle Command : Subsystem
  FMS_Out : Outport
  wires:
  Constant5/1 -> Data Type Conversion/1
  Heading Command/1(psi_rate_cmd_radPs) -> Bus Assignment/7
  Constant/1 -> Bus Assignment/1
  Attitude Command/1(phi_cmd_radPs) -> Bus Assignment/5
  Throttle Command/1(throttle_cmd) -> Bus Assignment/8
  Attitude Command/2(theta_cmd_radPs) -> Bus Assignment/6
  FMS_In/1 -> Attitude Command/1(FMS_In), Throttle Command/1(FMS_In), Heading Command/1(FMS_In)
  Bus Assignment/1 -> FMS_Out/1
  Data Type Conversion/1 -> Bus Assignment/2
  Constant1/1 -> Data Type Conversion1/1
  Data Type Conversion1/1 -> Bus Assignment/3
  Constant2/1 -> Data Type Conversion2/1
  Data Type Conversion2/1 -> Bus Assignment/4

== system FMS/FMS Commander/Commander/Arm/MC_Mode/Assist/Unknown ==
  Action Port : ActionPort  InitializeStates=reset  ActionType=default
  Bus Assignment : BusAssignment  AssignedSignals=reset,status,state,actuator_cmd
  Constant : Constant  Value=0  OutDataTypeStr=Bus: FMS_Out_Bus
  Constant1 : Constant  Value=VehicleStatus.Disarm
  Constant2 : Constant  OutDataTypeStr=Inherit: Inherit via back propagation
  Constant3 : Constant  Value=[1000;1000;1000;1000]  VectorParams1D=off  OutDataTypeStr=Inherit: Inherit via back propagation
  Constant4 : Constant  Value=zeros(12,1)  OutDataTypeStr=Inherit: Inherit via back propagation
  Constant5 : Constant  Value=VehicleState.Disarm
  Data Type Conversion : DataTypeConversion
  Data Type Conversion1 : DataTypeConversion
  Mux : Mux  Inputs=2
  FMS_Out : Outport
  wires:
  Mux/1 -> Bus Assignment/5
  Constant4/1 -> Mux/2
  Constant3/1 -> Mux/1
  Constant1/1 -> Data Type Conversion/1
  Constant2/1 -> Bus Assignment/2
  Bus Assignment/1 -> FMS_Out/1
  Constant/1 -> Bus Assignment/1
  Constant5/1 -> Data Type Conversion1/1
  Data Type Conversion/1 -> Bus Assignment/3
  Data Type Conversion1/1 -> Bus Assignment/4

== system FMS/FMS Commander/Commander/Arm/MC_Mode/Auto/Mission ==
  FMS_In : Inport
  Action Port : ActionPort  InitializeStates=reset  ActionType=case
      settings: CopyFcn=Stateflow.SLINSF.SimulinkMan.removeBlockPreDeleteFcn
  Bus Selector : BusSelector  OutputSignals=wp_index
  Detect Change : simulink/Logic and Bit Operations/Detect Change  vinit=0  OutDataTypeStr=boolean
  Mission_SubSystem : Subsystem  TreatAsAtomicUnit=on
  FMS_Out : Outport
  wires:
  Mission_SubSystem/1(FMS_Out) -> FMS_Out/1
  FMS_In/1 -> Bus Selector/1, Mission_SubSystem/1(FMS_In)
  Bus Selector/1 -> Detect Change/1  "<wp_index>"
  Detect Change/1 -> Mission_SubSystem/Reset

== system FMS/FMS Commander/Commander/Arm/MC_Mode/Auto/Offboard ==
  FMS_In : Inport
  Action Port : ActionPort  InitializeStates=reset  ActionType=case
      settings: CopyFcn=Stateflow.SLINSF.SimulinkMan.removeBlockPreDeleteFcn
  Acc_Command : Subsystem
  Bus Assignment : BusAssignment  AssignedSignals=status,state,ctrl_mode,p_cmd,q_cmd,r_cmd,phi_cmd,theta_cmd,throttle_cmd,ax_cmd,ay_cmd,az_cmd,psi_rate_cmd,u_cmd,v_cmd,w_cmd,cmd_mask
  Bus Selector : BusSelector  OutputSignals=Auto_Cmd.p_cmd,Auto_Cmd.q_cmd,Auto_Cmd.r_cmd,Auto_Cmd.phi_cmd,Auto_Cmd.theta_cmd,Auto_Cmd.throttle_cmd
  Command_Mask : Subsystem
  Constant : Constant  Value=0  OutDataTypeStr=Bus: FMS_Out_Bus
  Constant1 : Constant  Value=VehicleStatus.Arm
  Constant2 : Constant  Value=VehicleState.Offboard
  Constant3 : Constant  Value=ControlMode.Offboard
  Data Type Conversion : DataTypeConversion
  Data Type Conversion1 : DataTypeConversion
  Data Type Conversion2 : DataTypeConversion
  Heading_Command : Subsystem
  Velocity_Command : Subsystem
  FMS_Out : Outport
  wires:
  Bus Assignment/1 -> FMS_Out/1
  Constant/1 -> Bus Assignment/1
  Constant1/1 -> Data Type Conversion/1
  Data Type Conversion/1 -> Bus Assignment/2
  Constant2/1 -> Data Type Conversion1/1
  Data Type Conversion1/1 -> Bus Assignment/3
  Data Type Conversion2/1 -> Bus Assignment/4
  Constant3/1 -> Data Type Conversion2/1
  Bus Selector/1 -> Bus Assignment/5  "<p_cmd>"
  Bus Selector/2 -> Bus Assignment/6  "<q_cmd>"
  Bus Selector/3 -> Bus Assignment/7  "<r_cmd>"
  Bus Selector/4 -> Bus Assignment/8  "<phi_cmd>"
  Bus Selector/5 -> Bus Assignment/9  "<theta_cmd>"
  Velocity_Command/1(u_cmd) -> Bus Assignment/15
  Velocity_Command/2(v_cmd) -> Bus Assignment/16
  Velocity_Command/3(w_cmd) -> Bus Assignment/17
  Bus Selector/6 -> Bus Assignment/10  "<throttle_cmd>"
  Acc_Command/1(ax_C_cmd) -> Bus Assignment/11
  Acc_Command/2(ay_C_cmd) -> Bus Assignment/12
  Acc_Command/3(az_C_cmd) -> Bus Assignment/13
  Command_Mask/1(cmd_mask) -> Bus Assignment/18
  Heading_Command/1(psi_rate_cmd) -> Bus Assignment/14
  FMS_In/1 -> Acc_Command/1(FMS_In), Command_Mask/1(FMS_In), Velocity_Command/1(FMS_In), Heading_Command/1(FMS_In), Bus Selector/1

== system FMS/FMS Commander/Commander/Arm/MC_Mode/Auto/Unknown ==
  Action Port : ActionPort  InitializeStates=reset  ActionType=default
  Bus Assignment : BusAssignment  AssignedSignals=reset,status,state,actuator_cmd
  Constant : Constant  Value=0  OutDataTypeStr=Bus: FMS_Out_Bus
  Constant1 : Constant  Value=VehicleStatus.Disarm
  Constant2 : Constant  OutDataTypeStr=Inherit: Inherit via back propagation
  Constant3 : Constant  Value=[1000;1000;1000;1000]  VectorParams1D=off  OutDataTypeStr=Inherit: Inherit via back propagation
  Constant4 : Constant  Value=zeros(12,1)  OutDataTypeStr=Inherit: Inherit via back propagation
  Constant5 : Constant  Value=VehicleState.Disarm
  Data Type Conversion : DataTypeConversion
  Data Type Conversion1 : DataTypeConversion
  Mux : Mux  Inputs=2
  FMS_Out : Outport
  wires:
  Mux/1 -> Bus Assignment/5
  Constant4/1 -> Mux/2
  Constant3/1 -> Mux/1
  Constant1/1 -> Data Type Conversion/1
  Constant2/1 -> Bus Assignment/2
  Bus Assignment/1 -> FMS_Out/1
  Constant/1 -> Bus Assignment/1
  Constant5/1 -> Data Type Conversion1/1
  Data Type Conversion/1 -> Bus Assignment/3
  Data Type Conversion1/1 -> Bus Assignment/4

== system FMS/FMS Commander/Commander/Arm/MC_Mode/SubMode/Hold ==
  FMS_In : Inport
  Action Port : ActionPort  InitializeStates=reset  ActionType=case
      settings: CopyFcn=Stateflow.SLINSF.SimulinkMan.removeBlockPreDeleteFcn
  Altitude Hold : Subsystem
  Bus Assignment : BusAssignment  AssignedSignals=status,state,ctrl_mode,psi_rate_cmd,u_cmd,v_cmd,w_cmd
  Constant : Constant  Value=0  OutDataTypeStr=Bus: FMS_Out_Bus
  Constant1 : Constant  Value=VehicleState.Hold
  Constant2 : Constant  Value=ControlMode.POSCTL
  Constant5 : Constant  Value=VehicleStatus.Arm
  Data Type Conversion : DataTypeConversion
  Data Type Conversion1 : DataTypeConversion
  Data Type Conversion2 : DataTypeConversion
  Heading Hold : Subsystem
  Position Hold : Subsystem
  FMS_Out : Outport
  wires:
  Bus Assignment/1 -> FMS_Out/1
  Altitude Hold/1(w_cmd_mPs) -> Bus Assignment/8
  Constant/1 -> Bus Assignment/1
  Position Hold/1(u_cmd_mPs) -> Bus Assignment/6
  Constant5/1 -> Data Type Conversion/1
  Position Hold/2(v_cmd_mPs) -> Bus Assignment/7
  Heading Hold/1(psi_rate_cmd_radPs) -> Bus Assignment/5
  Data Type Conversion/1 -> Bus Assignment/2
  Constant1/1 -> Data Type Conversion1/1
  Data Type Conversion1/1 -> Bus Assignment/3
  Constant2/1 -> Data Type Conversion2/1
  Data Type Conversion2/1 -> Bus Assignment/4
  FMS_In/1 -> Heading Hold/1(FMS_In), Altitude Hold/1(FMS_In), Position Hold/1(FMS_In)

== system FMS/FMS Commander/Commander/Arm/MC_Mode/SubMode/Land ==
  FMS_In : Inport
  Action Port : ActionPort  InitializeStates=reset  ActionType=case
      settings: CopyFcn=Stateflow.SLINSF.SimulinkMan.removeBlockPreDeleteFcn
  Assist Land Speed : Subsystem
  Bus Assignment1 : BusAssignment  AssignedSignals=status,state,ctrl_mode,psi_rate_cmd,u_cmd,v_cmd,w_cmd
  Bus Selector : BusSelector  OutputSignals=Cmd_In.sp_waypoint
  Constant : Constant  Value=0  OutDataTypeStr=Inherit: Inherit via back propagation
  Constant1 : Constant  Value=0  OutDataTypeStr=Bus: FMS_Out_Bus
  Constant2 : Constant  Value=ControlMode.POSCTL
  Constant3 : Constant  Value=VehicleState.Land
  Constant6 : Constant  Value=VehicleStatus.Arm
  Data Type Conversion : DataTypeConversion
  Data Type Conversion1 : DataTypeConversion
  Data Type Conversion2 : DataTypeConversion
  Position Command : Subsystem
  Selector : Selector  InputPortWidth=3  IndexOptions=Index vector (dialog)  Indices=[1 2]  OutputSizes=1
  FMS_Out : Outport
  wires:
  Selector/1 -> Position Command/2(land_xy_R)
  Bus Assignment1/1 -> FMS_Out/1
  Constant1/1 -> Bus Assignment1/1
  Position Command/1(u_cmd_mPs) -> Bus Assignment1/6
  Position Command/2(v_cmd_mPs) -> Bus Assignment1/7
  Constant/1 -> Bus Assignment1/5
  Constant2/1 -> Data Type Conversion2/1
  Constant6/1 -> Data Type Conversion/1
  Data Type Conversion/1 -> Bus Assignment1/2
  Constant3/1 -> Data Type Conversion1/1
  Data Type Conversion1/1 -> Bus Assignment1/3
  Data Type Conversion2/1 -> Bus Assignment1/4
  Bus Selector/1 -> Selector/1  "<sp_waypoint>"
  FMS_In/1 -> Assist Land Speed/1(FMS_In), Position Command/1(FMS_In), Bus Selector/1
  Assist Land Speed/1(w_cmd_mPs) -> Bus Assignment1/8

== system FMS/FMS Commander/Commander/Arm/MC_Mode/SubMode/Return ==
  FMS_In : Inport
  Action Port : ActionPort  InitializeStates=reset  ActionType=case
      settings: CopyFcn=Stateflow.SLINSF.SimulinkMan.removeBlockPreDeleteFcn
  Bus Assignment1 : BusAssignment  AssignedSignals=status,state,ctrl_mode,u_cmd,v_cmd,w_cmd,psi_rate_cmd
  Constant1 : Constant  Value=VehicleState.Return
  Constant2 : Constant  Value=0  OutDataTypeStr=Bus: FMS_Out_Bus
  Constant3 : Constant  Value=ControlMode.POSCTL
  Constant6 : Constant  Value=VehicleStatus.Arm
  Data Type Conversion : DataTypeConversion
  Data Type Conversion1 : DataTypeConversion
  Data Type Conversion2 : DataTypeConversion
  Heading Commander : Subsystem
  L1 : Constant  Value=FMS_PARAM.L1  OutDataTypeStr=single
  Sum : Sum  Inputs=+-|
  Velocity Commander : Subsystem
  Way Points : Subsystem
  FMS_Out : Outport
  wires:
  Sum/1 -> Heading Commander/2(p1p2)
  Way Points/2(p2) -> Sum/1, Velocity Commander/2(p2)
  Way Points/3(p3) -> Velocity Commander/3(p3)
  L1/1 -> Velocity Commander/4(L1)
  Constant3/1 -> Data Type Conversion2/1
  Way Points/1(p1) -> Sum/2, Velocity Commander/1(p1)
  Constant2/1 -> Bus Assignment1/1
  Heading Commander/2(psi_rad_cmd) -> Bus Assignment1/8
  Bus Assignment1/1 -> FMS_Out/1
  Data Type Conversion/1 -> Bus Assignment1/2
  Constant6/1 -> Data Type Conversion/1
  Data Type Conversion1/1 -> Bus Assignment1/3
  Data Type Conversion2/1 -> Bus Assignment1/4
  Constant1/1 -> Data Type Conversion1/1
  FMS_In/1 -> Heading Commander/1(FMS_In), Velocity Commander/5(FMS_In), Way Points/1(FMS_In)
  Velocity Commander/1(u_cmd) -> Bus Assignment1/5
  Velocity Commander/2(v_cmd) -> Bus Assignment1/6
  Velocity Commander/3(w_cmd) -> Bus Assignment1/7
  Heading Commander/1(psi_err_rad) -> Velocity Commander/6(psi_err_rad)
